simulink model "ATOM_simple_planning_simulator"  (R2026a)
settings: Solver=ode4  StopTime=100  FixedStep=0.01
StopFcn:
  | % Put every new figure in the same MATLAB Figures window as a docked tab.
  | set(groot, 'defaultFigureWindowStyle', 'docked');
  | 
  | if exist('costmap_active', 'var') && ...
  |     exist('vehicle', 'var') && ...
  |     exist('parking_path', 'var') && ...
  |     ~isempty(parking_path)
  | 
  |      plotPlan(costmap_active, vehicle, parking_path);
  | 
  |  else
  | 
  |      warning('No valid parking path is available for plotting.');
  | 
  |  end
  | 
  |  PlotControllerReferences( ...
  |      out.controller_reference_log);
  | 
  |  PlotControllerTracking( ...
  |      out.controller_tracking_log);
  | 
model workspace (MAT data in the model file):
  vehicle : object (value not decoded)
symbols that are objects in the model workspace (value not decoded): vehicle
undefined symbols (not defined in the file): delta_f_LUT, gain4WS_LUT, k_ref_LUT, kappa_gain_BP, Ki, Kp, lateral, longitudinal, planning_validator, rr_gain_BP, rr_LUT, stanley, velocity_smoother
libraries: slpidlib x1
(part 5 of 8)

== matlab function ATOM_simple_planning_simulator/Parking Scenario2/Costmap generation: empty occupancy grid/MATLAB Function ==
  data: veh input; costmap output Bus: OccupancyGridBus; start_pose output; goal_pose output
function [costmap, start_pose, goal_pose] = costmapEmptyLot(veh) %#ok<INUSD>
%COSTMAPEMPTYLOT  Empty lot - no objects layer. The reference case:
% whatever the planner does here is forced by the turning radius alone,
% not by obstacles.
%
% veh is unused (no parked cars to size) but kept so all costmap blocks
% have identical ports and can be rewired freely.

persistent occ

res = 0.3;   W = 234;   H = 234;
origin_x = -(W/2)*res;
origin_y = -(H/2)*res;

if isempty(occ)
    [IX, IY] = meshgrid(0:W-1, 0:H-1);
    X = origin_x + IX*res;
    Y = origin_y + IY*res;

    lot_x = [-15  15  15 -15];
    lot_y = [-12 -12  12  12];
    occ = ones(H,W);
    occ(inpolygon(X, Y, lot_x, lot_y)) = 0;
end

start_pose = [-8, 0, 0];
goal_pose  = [ 0, 5, pi/2];

costmap.info.resolution           = res;
costmap.info.width                = uint32(W);
costmap.info.height               = uint32(H);
costmap.info.origin.position.x    = origin_x;
costmap.info.origin.position.y    = origin_y;
costmap.info.origin.position.z    = 0;
costmap.info.origin.orientation.x = 0;
costmap.info.origin.orientation.y = 0;
costmap.info.origin.orientation.z = 0;
costmap.info.origin.orientation.w = 1;
costmap.data                      = int8(occ*100);
end

== matlab function ATOM_simple_planning_simulator/Plot vehicle/SetStanleyTrajectory/Resample Trajectory ==
  data: trajectory_in input Bus: TrajectoryDataBus; trajectory_out output Bus: TrajectoryDataBus; resample_interval_dist input; nearest_seg_idx input; ego_offset_to_segment input
function trajectory_out = resampleTrajectoryByDistance( ...
    trajectory_in, ...
    resample_interval_dist, ...
    nearest_seg_idx, ...
    ego_offset_to_segment)


%% ============================================================
% RESAMPLE TRAJECTORY BY ARC LENGTH
%
% Equivalent to:
%
% MPCUtils::resampleMPCTrajectoryByDistance()
%
% Adapted for Stanley controller.
%
% Unlike MPC:
% - no MPCTrajectory conversion
% - no curvature resampling
% - no optimization variables
%
% The trajectory is directly interpolated in arc length.
%
% ATTENTION:
% 
% Resampling is not actuated in Simulink since in/out buses present fixed sizes.
% See NOTE at the end of this function.
%
% =============================================================


% N = length(trajectory_in.pose.position.x);
% 
% 
% if N < 2
% 
%     trajectory_out = trajectory_in;
%     return
% 
% end
% 
% 
% 
% %% ============================================================
% % Compute arc length
% % =============================================================
% 
% x = trajectory_in.pose.position.x;
% y = trajectory_in.pose.position.y;
% 
% 
% arc_length = zeros(N,1);
% 
% 
% for i = 2:N
% 
%     dx = x(i)-x(i-1);
%     dy = y(i)-y(i-1);
% 
%     arc_length(i)= ...
%         arc_length(i-1)+sqrt(dx^2+dy^2);
% 
% end
% 
% 
% 
% if isempty(arc_length)
% 
%     trajectory_out = trajectory_in;
%     return
% 
% end
% 
% 
% 
% %% ============================================================
% % Ego position along trajectory
% %
% % Equivalent to:
% %
% % input_arclength(nearest_seg_idx)
% % + ego_offset_to_segment
% %
% % =============================================================
% 
% 
% ego_s = arc_length(nearest_seg_idx) ...
%         + ego_offset_to_segment;
% 
% 
% ego_s = min(max(ego_s,0),arc_length(end));
% 
% 
% 
% %% ============================================================
% % Generate resampling points
% %
% % Same strategy as Autoware:
% % - backward from ego
% % - forward from ego
% %
% % =============================================================
% 
% 
% output_s = [];
% 
% 
% % backward direction
% 
% s = ego_s;
% 
% while s >= 0
% 
%     output_s = [s output_s]; %#ok<AGROW>
% 
%     s = s - resample_interval_dist;
% 
% end
% 
% 
% 
% % forward direction
% 
% s = ego_s + resample_interval_dist;
% 
% 
% while s < arc_length(end)
% 
%     output_s(end+1)=s; % #ok<AGROW>
% 
%     s = s + resample_interval_dist;
% 
% end
% 
% 
% 
% %% ============================================================
% % Interpolation
% % =============================================================
% 
% 
% x_new = interp1( ...
%     arc_length,...
%     x,...
%     output_s,...
%     'linear');
% 
% 
% 
% y_new = interp1( ...
%     arc_length,...
%     y,...
%     output_s,...
%     'linear');
% 
% 
% 
% z = trajectory_in.pose.position.z;
% 
% z_new = interp1( ...
%     arc_length,...
%     z,...
%     output_s,...
%     'linear');
% 
% 
% 
% %% ============================================================
% % Quaternion / yaw interpolation
% %
% % Stanley works with yaw.
% % Therefore interpolate yaw and rebuild quaternion.
% %
% % =============================================================
% 
% 
% yaw = QuaternionToYaw( ...
%     trajectory_in.pose.orientation.qx,...
%     trajectory_in.pose.orientation.qy,...
%     trajectory_in.pose.orientation.qz,...
%     trajectory_in.pose.orientation.qw);
% 
% 
% 
% % avoid discontinuity
% 
% yaw = unwrap(yaw);
% 
% 
% 
% yaw_new = interp1( ...
%     arc_length,...
%     yaw,...
%     output_s,...
%     'linear');
% 
% 
% 
% %% ============================================================
% % Velocity interpolation
% %
% % Autoware uses linear interpolation
% % =============================================================
% 
% 
% vel_new = interp1( ...
%     arc_length,...
%     trajectory_in.longitudinal_velocity_mps,...
%     output_s,...
%     'linear');
% 
% 
% 
% lat_vel_new = interp1( ...
%     arc_length,...
%     trajectory_in.lateral_velocity_mps,...
%     output_s,...
%     'linear');
% 
% 
% 
% acc_new = interp1( ...
%     arc_length,...
%     trajectory_in.acceleration_mps2,...
%     output_s,...
%     'linear');
% 
% 
% 
% %% ============================================================
% % Build output structure
% % =============================================================
% 
% 
% M = length(output_s);
% 
% 
% trajectory_out.pose.position.x = x_new;
% trajectory_out.pose.position.y = y_new;
% trajectory_out.pose.position.z = z_new;
% 
% 
% 
% [qx,qy,qz,qw] = yawToQuaternion(yaw_new);
% 
% 
% 
% trajectory_out.pose.orientation.qx = qx;
% trajectory_out.pose.orientation.qy = qy;
% trajectory_out.pose.orientation.qz = qz;
% trajectory_out.pose.orientation.qw = qw;
% 
% 
% 
% trajectory_out.longitudinal_velocity_mps = vel_new;
% 
% trajectory_out.lateral_velocity_mps = lat_vel_new;
% 
% trajectory_out.acceleration_mps2 = acc_new;
% 
% 
% 
% % steering values are kept
% 
% trajectory_out.front_wheel_angle_rad = ...
%     interp1( ...
%     arc_length,...
%     trajectory_in.front_wheel_angle_rad,...
%     output_s,...
%     'linear');
% 
% 
% trajectory_out.rear_wheel_angle_rad = ...
%     interp1( ...
%     arc_length,...
%     trajectory_in.rear_wheel_angle_rad,...
%     output_s,...
%     'linear');
% 
% 


%% ============================================================
% NOTE (Simulink Implementation)
%
% The trajectory resampling algorithm reported above is equivalent
% to the implementation adopted by Autoware.
%
% However, the main objective of the present work is the development
% and validation of the 4WS Stanley Controller rather than the
% trajectory preprocessing module.
%
% Since Simulink requires fixed-size bus signals, the resampled
% trajectory is not generated in the simulation model.
%
% The original input trajectory is therefore directly propagated to
% the controller, preserving its fixed dimension and avoiding the
% introduction of variable-length signals.
%
% Consequently, the following assignment overwrites the resampled
% trajectory computed above.
%
% ============================================================

trajectory_out = trajectory_in;

end

== matlab function ATOM_simple_planning_simulator/Plot vehicle/Plot vehicle Front reference frame ==
  settings: updateMethod=DISCRETE
  data: kinematic input Bus: KinematicStateBus; steer_front input double; steer_rear input double; veh input; traj input
function plotVehicleFront(kinematic, steer_front, steer_rear, veh, traj)

%% Vehicle parameters

L  = veh(3);
track = veh(4);

front_overhang = veh(5);
rear_overhang  = veh(6);
left_overhang = veh(7);
right_overhang = veh(8);

vehicle_length  = L + front_overhang + rear_overhang;
vehicle_width = track + left_overhang + right_overhang;

wheel_width = veh(2);
wheel_radius = veh(1);

%% Reference trajectory

x_ref = traj.pose.position.x;
y_ref = traj.pose.position.y;

yaw_ref = zeros(length(x_ref),1);


for i=1:length(x_ref)

    yaw_ref(i)=2*atan2(...
        traj.pose.orientation.qz(i),...
        traj.pose.orientation.qw(i));
end


%% Current kinematic state

x = kinematic.pose.position.x;
y = kinematic.pose.position.y;

qz = kinematic.pose.orientation.z;
qw = kinematic.pose.orientation.w;

yaw = 2*atan2(qz,qw);

vx = kinematic.twist.linear.x;

steer_front = steer_front;
steer_rear = steer_rear;

%% Position and orientation vehicle body

vehicle_body = [front_overhang vehicle_width/2;
                front_overhang -vehicle_width/2;
                -L-rear_overhang -vehicle_width/2;
                -L-rear_overhang vehicle_width/2;
                front_overhang vehicle_width/2];

R_body = [ cos(yaw) -sin(yaw)
    sin(yaw)  cos(yaw) ];

body_world = (R_body*vehicle_body')';

body_world(:,1)=body_world(:,1)+x;
body_world(:,2)=body_world(:,2)+y;


%% Position and orientation wheels

wheel_body = [wheel_radius  wheel_width/2
                wheel_radius -wheel_width/2
                -wheel_radius -wheel_width/2
                -wheel_radius  wheel_width/2
                wheel_radius  wheel_width/2];

FL = [0  track/2];
FR = [0 -track/2];
RL = [-L  track/2];
RR = [-L -track/2];

centers = [FL;
    FR;
    RL;
    RR];

centers = (R_body*centers')';

centers(:,1) = centers(:,1)+x;
centers(:,2) = centers(:,2)+y;

wheelFL = transformWheel(centers(1,:),steer_front,yaw,wheel_body);
wheelFR = transformWheel(centers(2,:),steer_front,yaw,wheel_body);
wheelRL = transformWheel(centers(3,:),steer_rear,yaw,wheel_body);
wheelRR = transformWheel(centers(4,:),steer_rear,yaw,wheel_body);



persistent hFig
persistent ax
persistent hBody
persistent hWheelFL
persistent hWheelFR
persistent hWheelRL
persistent hWheelRR
persistent hTrajectory
persistent TrajX
persistent TrajY
persistent hRefTraj 
persistent hArrow


if isempty(hBody)
    hFig = figure(13);
    clf

    ax = axes(hFig);

    hold(ax,'on')
    axis(ax,'equal')
    grid(ax,'on')


    xlabel(ax,'x [m]')
    ylabel(ax,'y [m]')

    hBody = plot(body_world(:,1),...
        body_world(:,2),...
        'k','LineWidth',2);

    hWheelFL = plot(wheelFL(:,1),...
        wheelFL(:,2),...
        'r','LineWidth',2);

    hWheelFR = plot(wheelFR(:,1),...
        wheelFR(:,2),...
        'r','LineWidth',2);

    hWheelRL = plot(wheelRL(:,1),...
        wheelRL(:,2),...
        'b','LineWidth',2);

    hWheelRR = plot(wheelRR(:,1),...
        wheelRR(:,2),...
        'b','LineWidth',2);

    TrajX = x;
    TrajY = y;

    hTrajectory = plot(TrajX,...
                       TrajY,...
                       'g','LineWidth',1);

    hRefTraj=plot(x_ref,y_ref,'b','LineWidth',2);

    step=5;

    hArrow=quiver(...
        x_ref(1:step:end),...
        y_ref(1:step:end),...
        cos(yaw_ref(1:step:end)),...
        sin(yaw_ref(1:step:end)),...
        0.5,...
        'r');

else

    set(hBody,...
        'XData',body_world(:,1),...
        'YData',body_world(:,2));

    set(hWheelFL,...
        'XData',wheelFL(:,1),...
        'YData',wheelFL(:,2));

    set(hWheelFR,...
        'XData',wheelFR(:,1),...
        'YData',wheelFR(:,2));

    set(hWheelRL,...
        'XData',wheelRL(:,1),...
        'YData',wheelRL(:,2));

    set(hWheelRR,...
        'XData',wheelRR(:,1),...
        'YData',wheelRR(:,2));

    TrajX(end+1) = x;
    TrajY(end+1) = y;

 
    set(hTrajectory,...
        'XData',TrajX,...
        'YData',TrajY);

    set(hRefTraj,...
        'XData',x_ref,...
        'YData',y_ref);

    

end

margin = 12;
xlim(ax, [x-margin x+margin])
ylim(ax, [y-margin y+margin])

% xlim([-20 20])
% ylim([-20 20])

drawnow limitrate
pause(0.01)


end

== matlab function ATOM_simple_planning_simulator/Plot vehicle/SetStanleyTrajectory/calcLongOffsetToSegment ==
  data: seg_idx input; ego_pose input; trajectory input Bus: TrajectoryDataBus; ego_offset_to_segment output
function ego_offset_to_segment = calcLongOffsetToSegment(seg_idx, ego_pose, trajectory)

ego_offset_to_segment = calcLongitudinalOffsetToSegment(trajectory, seg_idx, ego_pose);

end

== matlab function ATOM_simple_planning_simulator/Plot vehicle/SetStanleyTrajectory/findFirstNearestSegmentIndexWithSoftConstraints ==
  data: trajectory input; dist_threshold input; yaw_threshold input; nearest_seg_idx output; pose input
function nearest_seg_idx = findNearestSegmentIndexWithSoftConstraints( ...
    trajectory, dist_threshold, yaw_threshold, pose)


%% Step 1:
% Find nearest point index

nearest_idx = findFirstNearestIndexWithSoftConstraints( ...
    trajectory, ...
    pose, ...
    dist_threshold, ...
    yaw_threshold);


N = length(trajectory.pose.position.x);


%% Step 2:
% Convert point index into segment index

% First point
if nearest_idx == 1

    nearest_seg_idx = 1;
    return

end


% Last point
if nearest_idx == N

    nearest_seg_idx = N-1;
    return

end



%% Step 3:
% Determine whether ego lies before or after nearest point
%
% Equivalent to Autoware:
%
% signed_length =
% calcLongitudinalOffsetToSegment(points,
%                                 nearest_idx,
%                                 pose.position)


signed_length = calcLongitudinalOffsetToSegment( ...
    trajectory,...
    nearest_idx,...
    pose);



%% Step 4:
% Choose segment

if signed_length <= 0

    % ego is before nearest point
    %
    % Autoware:
    % return nearest_idx - 1;

    nearest_seg_idx = nearest_idx - 1;


else

    % ego is after nearest point
    %
    % Autoware:
    % return nearest_idx;

    nearest_seg_idx = nearest_idx;

end


end

== matlab function ATOM_simple_planning_simulator/velocity_smoother_node/MATLAB Function1 ==
  data: trajectory_input input; trajectory_output input; curvature input
function PlotSteeringRateVelocityLimit( ...
    trajectory_input, ...
    trajectory_output, ...
    curvature)

% PlotSteeringRateVelocityLimit
%
% Visualizes the velocity modification produced by the steering-rate
% velocity constraint.
%
% Equivalent to inspecting the difference between:
%
%   input.longitudinal_velocity_mps
%
% and:
%
%   output.longitudinal_velocity_mps
%
% after:
%
%   SmootherBase::applySteeringRateLimit()
%
% in Autoware.
%
%
% The steering-rate filter does not modify the trajectory geometry.
% It only reduces longitudinal velocity where the steering rate
% constraint is violated.
%
%
% Inputs
% -------
%
% trajectory_input:
%       Trajectory before ApplySteeringRateVelocityLimit()
%
%       Required fields:
%           trajectory.longitudinal_velocity_mps
%
%
% trajectory_output:
%       Trajectory after ApplySteeringRateVelocityLimit()
%
%       Required fields:
%           trajectory.longitudinal_velocity_mps
%
%
% curvature:
%       trajectory curvature [1/m]
%
%       Used only for visualization of curved regions.
%
%
% Output
% -------
%
% None
%
% Generates diagnostic plots:
%
%   - velocity before/after steering-rate constraint
%   - velocity reduction
%   - curvature profile


%% Extract velocities

vel_in = trajectory_input.longitudinal_velocity_mps;
vel_out = trajectory_output.longitudinal_velocity_mps;


N = length(vel_in);


if length(vel_out) ~= N
    error("Input and output trajectories have different lengths.");
end


%% Velocity variation

velocity_delta = vel_out - vel_in;


%% Plot velocity profile

persistent hVelIn hVelOut hCurvature hVelDelta1 hVelDelta2


if isempty(hVelIn)

    figure(14)
    hold on
    grid on

    hVelIn = plot( ...
        vel_in,...
        'LineWidth',1.5,...
        'DisplayName',"Input velocity");
    
    hVelOut = plot( ...
        vel_out,...
        '--',...
        'LineWidth',1.5,...
        'DisplayName',"After steering-rate limit");


    xlabel("Trajectory point index");
    ylabel("Longitudinal velocity [m/s]");
    
    title("Lateral acceleration velocity limitation");
    
    legend("Location","best");

else
    
    set(hVelIn, ...
        'YData', vel_in);
    
    set(hVelOut, ...
        'YData', vel_out);
end

%% Plot velocity reduction


if isempty(hVelDelta1)

    figure(15)
    hold on
    grid on

    hVelDelta1 = plot( ...
        velocity_delta,...
        'LineWidth',1.5);
    
    
    yline(0);
    
    
    xlabel("Trajectory point index");
    ylabel("\Delta velocity [m/s]");
    
    
    title("Velocity modification due to lateral acceleration constraint");

else

    set(hVelDelta1, ...
        'YData', velocity_delta);


end

drawnow limitrate

end

== matlab function ATOM_simple_planning_simulator/Lateral run()/CalculateStanley/getData/calculate curvature predicted/CalcTrajectoryCurvature ==
  data: trajectory input Bus: TrajectoryDataBus; curvature output; nearest_idx input; idx_dist input
function curvature = ComputeNearestCurvature( ...
    trajectory,...
    nearest_idx, idx_dist)


%% ============================================================
% COMPUTE NEAREST TRAJECTORY CURVATURE
%
% Equivalent to:
%
% autoware::motion_utils::calcTrajectoryCurvatureFrom3Points()
%
% Difference:
%
% - Autoware computes curvature for the whole trajectory
% - Here only the curvature at nearest_idx is required
%   for Stanley controller
%
% Inputs:
%
% trajectory:
%   Reference trajectory
%
% nearest_idx:
%   Nearest trajectory point index
%
% idx_dist:
%   Distance in samples used for three-point fitting
%
%
% Output:
%
% curvature:
%   Local trajectory curvature [1/m]
%
% ============================================================

N = length(trajectory.pose.position.x);



%% Check trajectory length

if N < 3

    curvature = 0;
    return

end



%% Clamp index

nearest_idx = max(1,min(nearest_idx,N));



%% Select three points
%
% Equivalent to Autoware:
%
% p0 = trajectory[i-idx_dist]
% p1 = trajectory[i]
% p2 = trajectory[i+idx_dist]
%
% ============================================================


idx_prev = nearest_idx - min(idx_dist, nearest_idx-1);

idx_next = nearest_idx + min(idx_dist, N-nearest_idx);



p0 = [
    trajectory.pose.position.x(idx_prev),...
    trajectory.pose.position.y(idx_prev)
];


p1 = [
    trajectory.pose.position.x(nearest_idx),...
    trajectory.pose.position.y(nearest_idx)
];


p2 = [
    trajectory.pose.position.x(idx_next),...
    trajectory.pose.position.y(idx_next)
];



%% Compute curvature

curvature = calc_curvature(p0,p1,p2);


end

== matlab function ATOM_simple_planning_simulator/Lateral run()/CalculateStanley/getData/calculate curvature predicted/ComputeIdxDist ==
  data: points_interval input; idx_dist output; vel_smoother input
function idx_dist = ComputeIdxDist( ...
    points_interval, ...
    vel_smoother)

% ComputeIdxDist
%
% Computes the point offset used for trajectory curvature estimation.
%
% The curvature is evaluated using three trajectory points separated by a
% fixed physical distance. Since the trajectory is sampled with a constant
% spatial interval (points_interval), this function converts the desired
% curvature calculation distance into the corresponding point index offset.
%
% In other words, idx_dist represents the number of trajectory points
% corresponding to the specified curvature calculation distance.
%
% Equivalent to the Autoware implementation:
%
% idx_dist = max(int(curvature_calculation_distance / points_interval), 1);

curvature_calculation_distance = vel_smoother(1);

idx_dist = max( ...
    floor(curvature_calculation_distance / points_interval), ...
    1);

== matlab function ATOM_simple_planning_simulator/Lateral run()/CalculateStanley/getData/calculate curvature predicted/ComputePointsInterval ==
  data: input_points_interval input; vel_smoother input; use_resampling input; points_interval output
function points_interval = computePointsInterval(input_points_interval, ...
    vel_smoother, use_resampling)

% Compute the trajectory points interval used for preprocessing.
%
% If resampling is enabled, a constant spatial interval is imposed.
% Otherwise, the original trajectory point spacing is preserved.

sample_ds = vel_smoother(3,1);

if use_resampling

    points_interval = sample_ds;

else

    points_interval = input_points_interval;

end

end

== matlab function ATOM_simple_planning_simulator/Lateral run()/CalculateStanley/VerifyStanleyStatus ==
  data: steering_cmd input; stanley_solved_status output boolean; reason output
function [stanley_solved_status, reason] = VerifyStanleyStatus(steering_cmd)

% reason codes:
% 0 = OK
% 1 = Steering command is NaN/Inf
%
% Attention: in Autoware, reason is a String type. Just Simulink struggles
% with it.

stanley_solved_status = true;
reason = uint8(0);

if ~isfinite(steering_cmd)
    stanley_solved_status = false;
    reason = uint8(1);
end

== matlab function ATOM_simple_planning_simulator/Lateral run()/MATLAB Function1 ==
  data: solved input; previous_status output; reason input; previous_status input; previous_reason input; previous_reason output
function [previous_status, previous_reason] = StanleyStatusManager( ...
    solved,...
    reason,...
    previous_status,...
    previous_reason)

% ATTENTION!!!
% In Autoware, stanley_solved_status (originally mpc_solved_status) 
% is a struct, where equivalently:
% - solved = stanley_solved_status.result
% - reason = stanley_solved_status.reason
%
% StanleyStatusManager here is not implemented since it doesn't change the
% implementation of the controller.

previous_status = solved;
previous_reason = reason;

== matlab function ATOM_simple_planning_simulator/Lateral run()/UpdateSteeringOffset ==
  settings: updateMethod=DISCRETE
  data: steering input; twist input Bus: TwistBus; wheel_base input; update_vel_threshold input; update_steer_threshold input; average_num input; offset_limit input; steering_offset output; veh input
function steering_offset = updateSteeringOffset( ...
    steering,...
    twist,...
    wheel_base,...
    update_vel_threshold,...
    update_steer_threshold,...
    average_num,...
    offset_limit, ...
    veh)


persistent offset_storage
persistent count
persistent current_offset

rear_steering_ratio = veh(29);

if isempty(offset_storage)

    offset_storage = zeros(average_num,1);
    count = 0;
    current_offset = 0;

end


%% Current vehicle state

vx = twist.linear.x;
yaw_rate = twist.angular.z;



%% Check if offset update is allowed

update_offset = ...
    abs(vx) > update_vel_threshold && ...
    abs(steering) < update_steer_threshold;



if update_offset


    %% Estimate steering from vehicle motion

    rear_steering = rear_steering_ratio * steering;

    steer_angle_est = atan( ...
        yaw_rate*wheel_base/vx + tan(rear_steering));



    %% Compute offset

    new_offset = steering - steer_angle_est;



    %% Circular buffer

    count = count + 1;


    if count <= average_num

        offset_storage(count) = new_offset;

    else

        % shift left

        offset_storage(1:end-1)=offset_storage(2:end);

        offset_storage(end)=new_offset;

    end



    %% Compute average

    valid_samples = min(count,average_num);

    current_offset = mean(offset_storage(1:valid_samples));


end



%% Saturation (Autoware getOffset)

steering_offset = min(max(current_offset,...
    -offset_limit),...
    offset_limit);

end

== matlab function ATOM_simple_planning_simulator/Lateral run()/CalculateStanley/getData/calcNearestPoseInterpStanley1 ==
  data: self_pose input Bus: KinematicStateBus; trajectory input Bus: TrajectoryDataBus; nearest_pose output Bus: PoseBusStanley; max_dist input; max_yaw input; nearest_idx output
function [nearest_pose,nearest_idx]  = calcNearestPoseInterpStanley( ...
    self_pose, ...
    trajectory, ...
    max_dist, ...
    max_yaw)


%% ============================================================
% CALC NEAREST POSE INTERPOLATION FOR STANLEY CONTROLLER
%
% Equivalent to:
%
% MPCUtils::calcNearestPoseInterp()
%
% Differences with MPC:
%
% - Input trajectory is directly Trajectory message
% - No MPCTrajectory conversion
% - No relative_time prediction
% - Reference is already transformed to FRONT AXLE
%
% The function returns the continuous closest pose of the
% front axle on the reference trajectory.
%
% ============================================================


N = length(trajectory.pose.position.x);



%% ============================================================
% Initialization for code generation
% ============================================================

nearest_pose = struct();

nearest_pose.position.x = 0;
nearest_pose.position.y = 0;
nearest_pose.orientation.x = 0;
nearest_pose.orientation.y = 0;
nearest_pose.orientation.z = 0;
nearest_pose.orientation.w = 0;

nearest_idx = 1;

% nearest_velocity = 0;



if N == 0

    return

end



%% ============================================================
% Step 1:
% Find nearest trajectory index
%
% Equivalent to:
%
% findFirstNearestIndexWithSoftConstraints()
%
% ============================================================


nearest_idx = findFirstNearestIndexWithSoftConstraints( ...
    trajectory,...
    self_pose,...
    max_dist,...
    max_yaw);



%% ============================================================
% Single point trajectory
%
% Equivalent Autoware:
%
% if traj.size()==1
%
% ============================================================


if N == 1

    nearest_pose.x = trajectory.pose.position.x(1);
    nearest_pose.y = trajectory.pose.position.y(1);

    nearest_pose.orientation.x = trajectory.pose.orientation.qx(1);
    nearest_pose.orientation.y = trajectory.pose.orientation.qy(1);
    nearest_pose.orientation.z = trajectory.pose.orientation.qz(1);
    nearest_pose.orientation.w = trajectory.pose.orientation.qw(1);

    % nearest_velocity = trajectory.longitudinal_velocity_mps(1);

    return

end



%% ============================================================
% Step 2:
% Determine interpolation segment
%
% Equivalent to:
%
% calcLongitudinalOffset()
%
% ============================================================


if nearest_idx == 1

    prev_idx = 1;
    next_idx = 2;


elseif nearest_idx == N

    prev_idx = N-1;
    next_idx = N;


else


    p_nearest = [
        trajectory.pose.position.x(nearest_idx)
        trajectory.pose.position.y(nearest_idx)
        ];


    p_next = [
        trajectory.pose.position.x(nearest_idx+1)
        trajectory.pose.position.y(nearest_idx+1)
        ];


    signed_length = calcLongitudinalOffset( ...
        p_nearest,...
        p_next,...
        [self_pose.pose.position.x self_pose.pose.position.y]');


    if signed_length <= 0

        prev_idx = nearest_idx-1;
        next_idx = nearest_idx;

    else

        prev_idx = nearest_idx;
        next_idx = nearest_idx+1;

    end

end



%% ============================================================
% Step 3:
% Linear interpolation
%
% Equivalent to:
%
% nearest_pose.position =
% (1-ratio)*prev + ratio*next
%
% ============================================================


p_prev = [
    trajectory.pose.position.x(prev_idx)
    trajectory.pose.position.y(prev_idx)
];


p_next = [
    trajectory.pose.position.x(next_idx)
    trajectory.pose.position.y(next_idx)
];



segment_length = norm(p_next-p_prev);



% avoid division by zero

if segment_length < 1e-5


    nearest_pose.position.x = trajectory.pose.position.x(nearest_idx);
    nearest_pose.position.y = trajectory.pose.position.y(nearest_idx);


    nearest_pose.orientation.x = trajectory.pose.orientation.qx(nearest_idx);
    nearest_pose.orientation.y = trajectory.pose.orientation.qy(nearest_idx);
    nearest_pose.orientation.z = trajectory.pose.orientation.qz(nearest_idx);
    nearest_pose.orientation.w = trajectory.pose.orientation.qw(nearest_idx);

    % nearest_velocity = trajectory.longitudinal_velocity_mps(nearest_idx);


    return

end



%% Projection of ego on segment

offset = calcLongitudinalOffset( ...
    p_prev,...
    p_next,...
    [self_pose.pose.position.x self_pose.pose.position.y]');


ratio = min(max(offset / segment_length,0),1);



%% Interpolated position

nearest_pose.position.x = ...
    (1-ratio)*p_prev(1)+ratio*p_next(1);


nearest_pose.position.y = ...
    (1-ratio)*p_prev(2)+ratio*p_next(2);



%% ============================================================
% Yaw interpolation
%
% Equivalent:
%
% normalize_radian()
%
% ============================================================


yaw_prev = QuaternionToYaw( ...
    trajectory.pose.orientation.qx(prev_idx),...
    trajectory.pose.orientation.qy(prev_idx),...
    trajectory.pose.orientation.qz(prev_idx),...
    trajectory.pose.orientation.qw(prev_idx));


yaw_next = QuaternionToYaw( ...
    trajectory.pose.orientation.qx(next_idx),...
    trajectory.pose.orientation.qy(next_idx),...
    trajectory.pose.orientation.qz(next_idx),...
    trajectory.pose.orientation.qw(next_idx));


yaw_error = wrapToPi(yaw_prev-yaw_next);


nearest_yaw = wrapToPi( ...
    yaw_next + (1-ratio)*yaw_error);

[qx,qy,qz,qw] = yawToQuaternion(nearest_yaw);

nearest_pose.orientation.x = qx;
nearest_pose.orientation.y = qy;
nearest_pose.orientation.z = qz;
nearest_pose.orientation.w = qw;



% %% ============================================================
% % Velocity interpolation
% %
% % Stanley adaptation:
% %
% % The velocity is used for:
% % - gain scheduling
% % - softening factor
% %
% % ============================================================
% 
% 
% v_prev = trajectory.longitudinal_velocity_mps(prev_idx);
% 
% v_next = trajectory.longitudinal_velocity_mps(next_idx);
% 
% 
% nearest_velocity = ...
%     (1-ratio)*v_prev + ratio*v_next;


end

== matlab function ATOM_simple_planning_simulator/Lateral run()/CalculateStanley/getData/calculate curvature current/CalcTrajectoryCurvature ==
  data: trajectory input Bus: TrajectoryDataBus; curvature output; nearest_idx input; idx_dist input
function curvature = ComputeNearestCurvature( ...
    trajectory,...
    nearest_idx, idx_dist)


%% ============================================================
% COMPUTE NEAREST TRAJECTORY CURVATURE
%
% Equivalent to:
%
% autoware::motion_utils::calcTrajectoryCurvatureFrom3Points()
%
% Difference:
%
% - Autoware computes curvature for the whole trajectory
% - Here only the curvature at nearest_idx is required
%   for Stanley controller
%
% Inputs:
%
% trajectory:
%   Reference trajectory
%
% nearest_idx:
%   Nearest trajectory point index
%
% idx_dist:
%   Distance in samples used for three-point fitting
%
%
% Output:
%
% curvature:
%   Local trajectory curvature [1/m]
%
% ============================================================

N = length(trajectory.pose.position.x);



%% Check trajectory length

if N < 3

    curvature = 0;
    return

end



%% Clamp index

nearest_idx = max(1,min(nearest_idx,N));



%% Select three points
%
% Equivalent to Autoware:
%
% p0 = trajectory[i-idx_dist]
% p1 = trajectory[i]
% p2 = trajectory[i+idx_dist]
%
% ============================================================


idx_prev = nearest_idx - min(idx_dist, nearest_idx-1);

idx_next = nearest_idx + min(idx_dist, N-nearest_idx);



p0 = [
    trajectory.pose.position.x(idx_prev),...
    trajectory.pose.position.y(idx_prev)
];


p1 = [
    trajectory.pose.position.x(nearest_idx),...
    trajectory.pose.position.y(nearest_idx)
];


p2 = [
    trajectory.pose.position.x(idx_next),...
    trajectory.pose.position.y(idx_next)
];



%% Compute curvature

curvature = calc_curvature(p0,p1,p2);


end

== matlab function ATOM_simple_planning_simulator/Plot vehicle/Plot Vehicle Rear reference frame ==
  settings: updateMethod=DISCRETE
  data: kinematic input Bus: KinematicStateBus; steer_front input double; steer_rear input double; veh input; traj input
function plotVehicleRear(kinematic, steer_front, steer_rear, veh, traj)

%% Vehicle parameters

L  = veh(3);
track = veh(4);

front_overhang = veh(5);
rear_overhang  = veh(6);
left_overhang = veh(7);
right_overhang = veh(8);

vehicle_length  = L + front_overhang + rear_overhang;
vehicle_width = track + left_overhang + right_overhang;

wheel_width = veh(2);
wheel_radius = veh(1);

%% Reference trajectory

x_ref = traj.pose.position.x;
y_ref = traj.pose.position.y;


%% Current kinematic state

x = kinematic.pose.position.x;
y = kinematic.pose.position.y;

qz = kinematic.pose.orientation.z;
qw = kinematic.pose.orientation.w;

yaw = 2*atan2(qz,qw);

vx = kinematic.twist.linear.x;

steer_front = steer_front;
steer_rear = steer_rear;

%% Position and orientation vehicle body

vehicle_body = [L+front_overhang vehicle_width/2;
                L+front_overhang -vehicle_width/2;
                -rear_overhang -vehicle_width/2;
                -rear_overhang vehicle_width/2;
                L+front_overhang vehicle_width/2];

R_body = [ cos(yaw) -sin(yaw)
    sin(yaw)  cos(yaw) ];

body_world = (R_body*vehicle_body')';

body_world(:,1)=body_world(:,1)+x;
body_world(:,2)=body_world(:,2)+y;


%% Position and orientation wheels

wheel_body = [wheel_radius  wheel_width/2
                wheel_radius -wheel_width/2
                -wheel_radius -wheel_width/2
                -wheel_radius  wheel_width/2
                wheel_radius  wheel_width/2];

FL = [L  track/2];
FR = [L -track/2];
RL = [0  track/2];
RR = [0 -track/2];

centers = [FL;
    FR;
    RL;
    RR];

centers = (R_body*centers')';

centers(:,1) = centers(:,1)+x;
centers(:,2) = centers(:,2)+y;

wheelFL = transformWheel(centers(1,:),steer_front,yaw,wheel_body);
wheelFR = transformWheel(centers(2,:),steer_front,yaw,wheel_body);
wheelRL = transformWheel(centers(3,:),steer_rear,yaw,wheel_body);
wheelRR = transformWheel(centers(4,:),steer_rear,yaw,wheel_body);



persistent hFig
persistent ax
persistent hBody
persistent hWheelFL
persistent hWheelFR
persistent hWheelRL
persistent hWheelRR
persistent hTrajectory
persistent TrajX
persistent TrajY
persistent hRefTraj 


if isempty(hBody)
    hFig = figure(1);
    clf

    ax = axes(hFig);

    hold(ax,'on')
    axis(ax,'equal')
    grid(ax,'on')


    xlabel(ax,'x [m]')
    ylabel(ax,'y [m]')

    hBody = plot(body_world(:,1),...
        body_world(:,2),...
        'k','LineWidth',2);

    hWheelFL = plot(wheelFL(:,1),...
        wheelFL(:,2),...
        'r','LineWidth',2);

    hWheelFR = plot(wheelFR(:,1),...
        wheelFR(:,2),...
        'r','LineWidth',2);

    hWheelRL = plot(wheelRL(:,1),...
        wheelRL(:,2),...
        'b','LineWidth',2);

    hWheelRR = plot(wheelRR(:,1),...
        wheelRR(:,2),...
        'b','LineWidth',2);

    TrajX = x;
    TrajY = y;

    hTrajectory = plot(TrajX,...
                       TrajY,...
                       'g','LineWidth',1);

    hRefTraj=plot(x_ref,y_ref,'b','LineWidth',2);

else

    set(hBody,...
        'XData',body_world(:,1),...
        'YData',body_world(:,2));

    set(hWheelFL,...
        'XData',wheelFL(:,1),...
        'YData',wheelFL(:,2));

    set(hWheelFR,...
        'XData',wheelFR(:,1),...
        'YData',wheelFR(:,2));

    set(hWheelRL,...
        'XData',wheelRL(:,1),...
        'YData',wheelRL(:,2));

    set(hWheelRR,...
        'XData',wheelRR(:,1),...
        'YData',wheelRR(:,2));

    TrajX(end+1) = x;
    TrajY(end+1) = y;

 
    set(hTrajectory,...
        'XData',TrajX,...
        'YData',TrajY);

    set(hRefTraj,...
        'XData',x_ref,...
        'YData',y_ref);

end

margin = 12;
xlim(ax, [x-margin x+margin])
ylim(ax, [y-margin y+margin])

% xlim([-20 20])
% ylim([-20 20])

drawnow limitrate
pause(0.01)


end

== matlab function ATOM_simple_planning_simulator/Lateral run()/CalculateStanley/getData/calculate curvature current/ComputeIdxDist ==
  data: points_interval input; idx_dist output; vel_smoother input
function idx_dist = ComputeIdxDist( ...
    points_interval, ...
    vel_smoother)

% ComputeIdxDist
%
% Computes the point offset used for trajectory curvature estimation.
%
% The curvature is evaluated using three trajectory points separated by a
% fixed physical distance. Since the trajectory is sampled with a constant
% spatial interval (points_interval), this function converts the desired
% curvature calculation distance into the corresponding point index offset.
%
% In other words, idx_dist represents the number of trajectory points
% corresponding to the specified curvature calculation distance.
%
% Equivalent to the Autoware implementation:
%
% idx_dist = max(int(curvature_calculation_distance / points_interval), 1);

curvature_calculation_distance = vel_smoother(1);

idx_dist = max( ...
    floor(curvature_calculation_distance / points_interval), ...
    1);

== matlab function ATOM_simple_planning_simulator/Lateral run()/CalculateStanley/getData/calculate curvature current/ComputePointsInterval ==
  data: input_points_interval input; vel_smoother input; use_resampling input; points_interval output
function points_interval = computePointsInterval(input_points_interval, ...
    vel_smoother, use_resampling)

% Compute the trajectory points interval used for preprocessing.
%
% If resampling is enabled, a constant spatial interval is imposed.
% Otherwise, the original trajectory point spacing is preserved.

sample_ds = vel_smoother(3,1);

if use_resampling

    points_interval = sample_ds;

else

    points_interval = input_points_interval;

end

end

== matlab function ATOM_simple_planning_simulator/Lateral run()/CalculateStanley/RearToFrontOdometry ==
  data: rear_pose input Bus: KinematicStateBus; front_pose_pred output Bus: KinematicStateBus; wheel_base input
function front_pose_pred = RearToFrontOdometryCurrent( ...
    rear_pose, ...
    wheel_base)

front_pose_pred = rear_pose;

% 1. Estrazione dello Yaw dall'orientamento (Quaternion -> Yaw)
qx = rear_pose.pose.orientation.x;
qy = rear_pose.pose.orientation.y;
qz = rear_pose.pose.orientation.z;
qw = rear_pose.pose.orientation.w;
yaw = QuaternionToYaw(qx, qy, qz, qw);

% 2. Calcolo della Posizione Attuale dell'Asse Anteriore (Mappa/World Frame)
x_front_now = rear_pose.pose.position.x + wheel_base * cos(yaw);
y_front_now = rear_pose.pose.position.y + wheel_base * sin(yaw);

% 3. Velocità dell'Asse Anteriore espresso nel Frame Veicolo (Body Frame)
v_x_body = rear_pose.twist.linear.x;
v_y_body = rear_pose.twist.linear.y + rear_pose.twist.angular.z * wheel_base;

% 4. Conversione delle Velocità dal Frame Veicolo (Body) al Frame Mappa (World)
% Ruotiamo il vettore velocità [v_x_body, v_y_body] dell'angolo yaw attuale:
v_x_world = v_x_body * cos(yaw) - v_y_body * sin(yaw);
v_y_world = v_x_body * sin(yaw) + v_y_body * cos(yaw);

% 5. PREDIZIONE TEMPORALE (Coordinate t + tau nel Frame Mappa)
front_pose_pred.pose.position.x = x_front_now;
front_pose_pred.pose.position.y = y_front_now;
front_pose_pred.pose.position.z = rear_pose.pose.position.z;

% 6. Aggiornamento delle velocità nel messaggio di output (Frame Veicolo)
front_pose_pred.twist.linear.x = v_x_body;
front_pose_pred.twist.linear.y = v_y_body;
front_pose_pred.twist.linear.z = rear_pose.twist.linear.z;

% 7. L'orientamento rimane lo stesso (o aggiornato con il pitch/roll se presente)
front_pose_pred.pose.orientation = rear_pose.pose.orientation;

end

== matlab function ATOM_simple_planning_simulator/Lateral run()/CalculateStanley/getData/ChooseCurvature ==
  data: curvature_pred input; curvature output; curvature_curr input
function curvature = ChooseCurvature(curvature_pred, curvature_curr)

% =========================================
%
% Left turns: curvature > 0
% Right turns: curvature < 0
%
% =========================================

curvature_max = sin(2*0.7)/(2*cos(-0.7));

if abs(curvature_pred) >= abs(curvature_curr)
    if abs(curvature_pred) >= curvature_max
        sign_k = sign(curvature_pred);
        curvature = sign_k*curvature_max;
    else
        curvature = curvature_pred;
    end
else
    if abs(curvature_curr) >= curvature_max
        sign_k = sign(curvature_curr);
        curvature = sign_k*curvature_max;
    else
        curvature = curvature_curr;
    end


end

== matlab function ATOM_simple_planning_simulator/Lateral run()/Adaptive d0 ==
  data: d0 output; tau_steer input
function d0 = ComputeAdaptived0(tau_steer)

% d0 is the distance ahead of the vehicle, necessary for prediction.
% It's independent from current vehicle speed.
% We've seen that with time_constant = 0.27 --> d0 = 0.3.

d0 = (0.3/0.27)*tau_steer;

end

== matlab function ATOM_simple_planning_simulator/Lane Follower Scenario/Demanded trajectory generation: Serpentine/Trajectory Generator: 90° left turn critical for 2WS ==
  data: x output; y output; z output; qx output; qy output; qz output; qw output; longitudinal_velocity_mps output; lateral_velocity_mps output; acceleration_mps2 output; heading_rate_rps output; front_wheel_angle_rad output; rear_wheel_angle_rad output
function [x,y,z,qx,qy,qz,qw,...
          longitudinal_velocity_mps,...
          lateral_velocity_mps,...
          acceleration_mps2,...
          heading_rate_rps,...
          front_wheel_angle_rad,...
          rear_wheel_angle_rad] = trajectoryGenerator

N = 100;

%% Geometry

R = 3;                  % Radius [m]

N1 = 20;                % First straight
N2 = 30;                % Left curve
N3 = 30;                % Right curve
N4 = 20;                % Final straight


%% Allocate outputs

x = zeros(N,1);
y = zeros(N,1);
z = zeros(N,1);

qx = zeros(N,1);
qy = zeros(N,1);
qz = zeros(N,1);
qw = zeros(N,1);

longitudinal_velocity_mps = 6/3.6 * ones(N,1);

lateral_velocity_mps = zeros(N,1);
acceleration_mps2 = zeros(N,1);
heading_rate_rps = zeros(N,1);

front_wheel_angle_rad = zeros(N,1);
rear_wheel_angle_rad = zeros(N,1);


%% ========================================================================
%% First straight
%% ========================================================================

L1 = 2;

for i = 1:N1

    t = (i-1)/(N1-1);

    x(i) = t*L1;
    y(i) = 0;

    yaw = 0;

    qz(i) = sin(yaw/2);
    qw(i) = cos(yaw/2);

end


%% ========================================================================
%% First curve (LEFT)
%% ========================================================================

center1_x = L1;
center1_y = R;

theta = linspace(-pi/2,0,N2);

for k = 1:N2

    i = N1 + k;

    x(i) = center1_x + R*cos(theta(k));
    y(i) = center1_y + R*sin(theta(k));

    yaw = theta(k) + pi/2;

    qz(i) = sin(yaw/2);
    qw(i) = cos(yaw/2);

end


%% ========================================================================
%% Second curve (RIGHT)
%% Tangent to the previous one
%% ========================================================================

x_join = x(N1+N2);
y_join = y(N1+N2);

center2_x = x_join + R;
center2_y = y_join;

theta = linspace(pi,pi/2,N3);

for k = 1:N3

    i = N1 + N2 + k;

    x(i) = center2_x + R*cos(theta(k));
    y(i) = center2_y + R*sin(theta(k));

    yaw = theta(k) - pi/2;

    qz(i) = sin(yaw/2);
    qw(i) = cos(yaw/2);

end


%% ========================================================================
%% Final straight
%% ========================================================================

L2 = 15;

x0 = x(N1+N2+N3);
y0 = y(N1+N2+N3);

for k = 1:N4

    i = N1 + N2 + N3 + k;

    t = k/N4;

    x(i) = x0 + t*L2;
    y(i) = y0;

    yaw = 0;

    qz(i) = sin(yaw/2);
    qw(i) = cos(yaw/2);

end

end

== matlab function ATOM_simple_planning_simulator/LongitudinalRun()/nearest_idx ==
  data: trajectory input; nearest_idx output; self_pose input; max_dist input; max_yaw input
function nearest_idx = findFirstNearestIndexWithSoftConstraints(trajectory, self_pose, max_dist, max_yaw)

nearest_idx = findFirstNearestIndexWithSoftConstraints( ...
    trajectory,...
    self_pose,...
    max_dist,...
    max_yaw);

end

== matlab function ATOM_simple_planning_simulator/velocity_smoother_node/ApplyLateralAccelerationFilter - velocity_smoother node/ComputeVelocityProfile and Acceleration ==
  data: a_accel_max input; a_decel_max input; v_start input; v_end input; trajectory output; trajectory input Bus: TrajectoryDataBus
function trajectory = ComputeVelocityProfile( ...
    a_accel_max, a_decel_max, v_start, v_end, trajectory)
%% This function is mainly to calculate the longitudinal velocity and acceleration profile of
%%on the trajectory in order to be in the output trajectory bus of the velocity smoother block
%%going to the vehicle model

N  = length(trajectory.longitudinal_velocity_mps);
px = trajectory.pose.position.x;
py = trajectory.pose.position.y;

%% Pass 1: arc-length spacing between consecutive points
ds = zeros(N-1,1);
for i = 1:N-1
    ds(i) = sqrt( (px(i+1)-px(i))^2 + (py(i+1)-py(i))^2 );
end

%% Pass 2: backward - deceleration feasibility
% Answers: how fast can I be here and still slow down for what's ahead?
v_bwd    = trajectory.longitudinal_velocity_mps;   % ceiling from prior stages
v_bwd(N) = min(v_bwd(N), v_end);
for i = N-1:-1:1
    v_reach  = sqrt( v_bwd(i+1)^2 + 2*a_decel_max*ds(i) );
    v_bwd(i) = min( v_bwd(i), v_reach );
end

%% Pass 3: forward - acceleration feasibility
% Answers: how fast can I actually have gotten to here?
v    = v_bwd;
v(1) = min( v_bwd(1), v_start );
for i = 2:N
    v_reach = sqrt( v(i-1)^2 + 2*a_accel_max*ds(i-1) );
    v(i)    = min( v_bwd(i), v_reach );
end

%% Extract acceleration from the finished profile
a = zeros(N,1);
for i = 1:N-1
    if ds(i) > 1e-6
        a(i) = ( v(i+1)^2 - v(i)^2 ) / ( 2*ds(i) );
    else
        a(i) = 0;      % zero-length segment guard
    end
end
a(N) = 0;              % no segment ahead of the last point

trajectory.longitudinal_velocity_mps = v;
trajectory.acceleration_mps2         = a;
end

== matlab function ATOM_simple_planning_simulator/velocity_smoother_node/ApplyLateralAccelerationFilter - velocity_smoother node/MATLAB Function1 ==
  data: a_lat_max input; trajectory output; min_curve_velocity input; curvature input; trajectory input Bus: TrajectoryDataBus
function trajectory  = ApplyLateralAccelerationLimit( ...
    a_lat_max, min_curve_velocity, curvature, trajectory)
% Limits trajectory velocity so that lateral acceleration v^2/R
% never exceeds a_lat_max.
%
% Equivalent to SmootherBase::applyLateralAccelerationFilter() in Autoware,
% minus the decel_distance_before/after_curve ramps - those are unnecessary
% here because ComputeVelocityProfile's backward pass already produces the
% early ramp-down from first principles.

N = length(trajectory.longitudinal_velocity_mps);

for i = 1:N

    k = abs(curvature(i));
    delta_r = trajectory.rear_wheel_angle_rad(i);

    % Straight segment: no lateral constraint
    if k < 1e-6
        continue
    end
    %given a limit and a corner, what's the fastest you can go?
    % v_max such that v^2 * k <= a_lat_max
    v_lat_max = sqrt(a_lat_max*cos(delta_r)/ k);

    % Floor, so tight curves don't demand a crawl
    v_lat_max = max(v_lat_max, min_curve_velocity);

    % Can only lower the ceiling, never raise it
    trajectory.longitudinal_velocity_mps(i) = ...
        min(trajectory.longitudinal_velocity_mps(i), v_lat_max);
end
fprintf('kappa max %.4f | v ceiling [%.2f %.2f]\n', ...
    max(abs(curvature)), min(trajectory.longitudinal_velocity_mps), ...
    max(trajectory.longitudinal_velocity_mps));
end

== matlab function ATOM_simple_planning_simulator/Vehicle Model/localization//acceleration function ==
  data: state input Bus: VehicleInternalStateBus; accel output Bus: AccelerationBus; veh input
function accel = IntStateToAccelerationState(state,veh)

L = veh(3);

vx = state.vx;
ax = state.acc;

delta_f = state.steer_front;
delta_r = state.steer_rear;

yaw_rate = (vx/L)*(tan(delta_f)-tan(delta_r));

ay = vx*yaw_rate;

accel.acceleration.linear.x = ax;
accel.acceleration.linear.y = ay;
accel.acceleration.linear.z = 0;

accel.acceleration.angular.x = 0;
accel.acceleration.angular.y = 0;
accel.acceleration.angular.z = 0;

end
